simulink model "Sistema1"  (R2026a)
settings: Solver=ode15s  StopTime=20  MaxStep=0.01  RelTol=1e-6
libraries: fl_lib x18, nesl_utility x6, slpidlib x1
settings Model: Creator=sarag  LastModifiedBy=emivilg
settings DataIOCC: TimeSaveName=t
settings SimscapeCC: SimscapeNominalValues="[{\"value\":\"1\",\"unit\":\"A\"},{\"value\":\"1\",\"unit\":\"bar\"},{\"value\":\"1\",\"unit\":\"cm^2\"},{\"value\":\"1\",\"unit\":\"cm^3/s\"},{\"value\":\"1\",\"unit\":\"kJ/kg\"},{\"value\":\"1\",\"unit\":\"kW\"},{\"value\":\"1\",\"unit\":\"l\"},{\"value\":\"1\",\"unit\":\"N\"},{\"value\":\"1\",\"unit\":\"N*m\"},{\"value\":\"1\",\"unit\":\"V\"}]"  SimscapeLogType=none  SimscapeLogDataHistory=5000.0

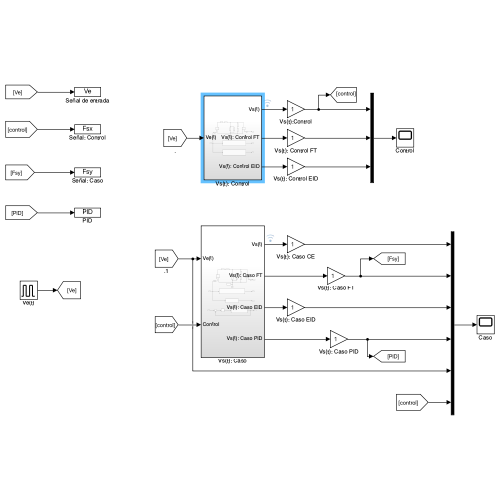
[thumbnail: Simulink's stored preview of the top-level diagram]
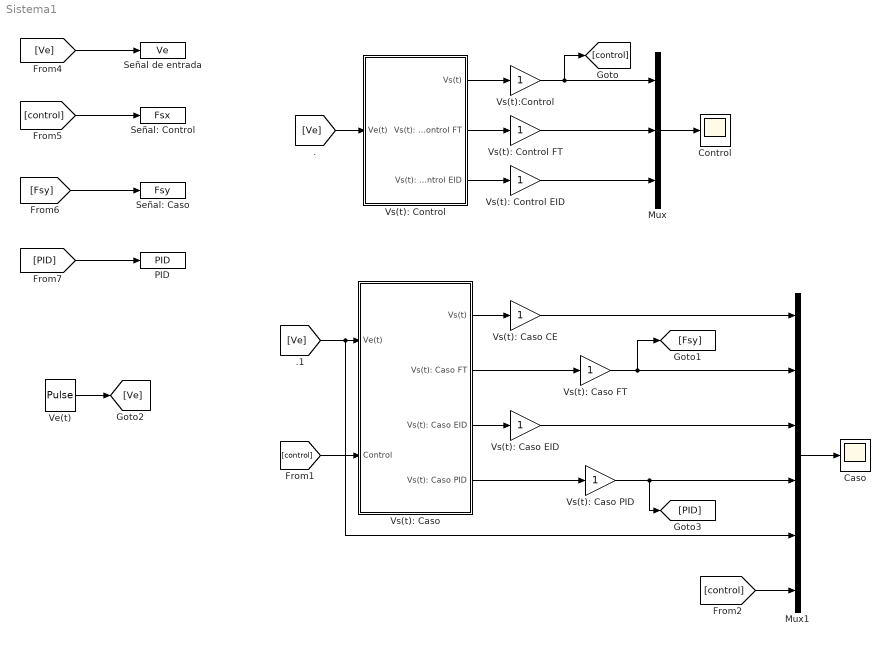
== system Sistema1 ==
  Caso : Scope
      settings: ActiveDisplayYMinimum=-0.12376243766517554  ActiveDisplayYMaximum=1.1138614462905658
  Control : Scope
      settings: ActiveDisplayYMinimum=-0.12361899608688497  ActiveDisplayYMaximum=1.112570964781965
  Mux : Mux  Inputs=3
  Mux1 : Mux  Inputs=6
  PID : ToWorkspace  VariableName=PID  SampleTime=-1
  Señal de entrada : ToWorkspace  VariableName=Ve  SampleTime=-1
  Señal: Caso : ToWorkspace  VariableName=Fsy  SampleTime=-1
  Señal: Control : ToWorkspace  VariableName=Fsx  SampleTime=-1
  Ve(t) : DiscretePulseGenerator  PulseType=Time based  Period=10  PulseWidth=5
  Vs(t): Caso : Subsystem
  Vs(t): Caso CE : Gain
  Vs(t): Caso EID : Gain
  Vs(t): Caso FT : Gain
  Vs(t): Caso PID : Gain
  Vs(t): Control : Subsystem
  Vs(t): Control EID : Gain
  Vs(t): Control FT : Gain
  Vs(t):Control : Gain
  wires:
  Mux/1 -> Control/1
  [Ve] -> Vs(t): Control/1(Ve(t))
  Vs(t): Control/1(Vs(t)) -> Vs(t):Control/1
  Vs(t): Caso/1(Vs(t)) -> Vs(t): Caso CE/1
  Vs(t): Caso/2(Vs(t): Caso FT) -> Vs(t): Caso FT/1
  Vs(t): Caso/3(Vs(t): Caso EID) -> Vs(t): Caso EID/1
  Vs(t): Caso/4(Vs(t): Caso PID) -> Vs(t): Caso PID/1
  Mux1/1 -> Caso/1
  Vs(t): Control/2(Vs(t): Control FT) -> Vs(t): Control FT/1
  Vs(t): Control/3(Vs(t): Control EID) -> Vs(t): Control EID/1
  Ve(t)/1 -> [Ve]
  [PID] -> PID/1
  [Fsy] -> Señal: Caso/1
  [control] -> Señal: Control/1
  [Ve] -> Señal de entrada/1
  Vs(t):Control/1 -> [control], Mux/1
  Vs(t): Control EID/1 -> Mux/3
  Vs(t): Caso CE/1 -> Mux1/1
  Vs(t): Caso FT/1 -> [Fsy], Mux1/2
  Vs(t): Caso EID/1 -> Mux1/3
  Vs(t): Caso PID/1 -> [PID], Mux1/4
  [control] -> Vs(t): Caso/2(Control)
  Vs(t): Control FT/1 -> Mux/2
  [control] -> Mux1/6
  [Ve] -> Mux1/5, Vs(t): Caso/1(Ve(t))

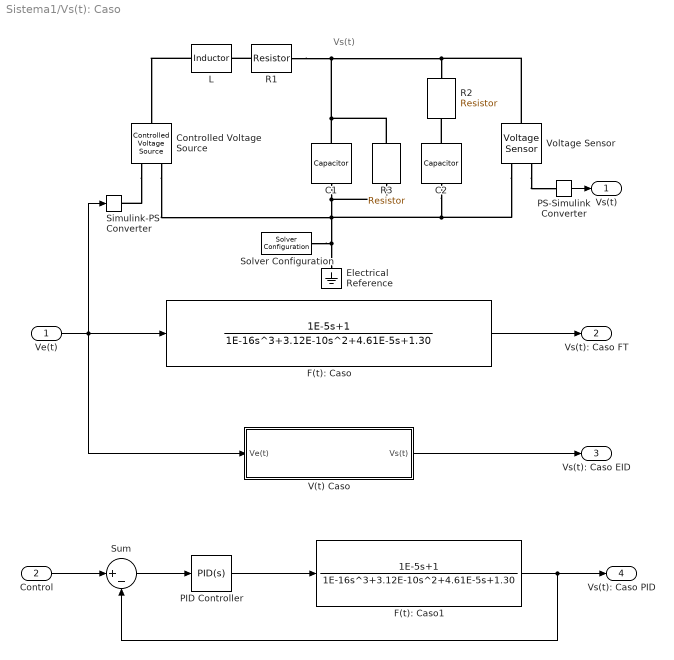
== system Sistema1/Vs(t): Caso ==
  note: Vs(t)
  Ve(t) : Inport
  Control : Inport  Port=2
  C1 : fl_lib/Electrical/Electrical Elements/Capacitor  c=1 uF  r=1e-6 Ohm  g=0 1/Ohm  i_specify=off  i_priority=None  i=0 A  i_nominal_specify=off  i_nominal_value=1  i_nominal_unit=A  v_specify=off  v_priority=None  v=0 V  v_nominal_specify=off  v_nominal_value=1  v_nominal_unit=V  vc_specify=off  vc_priority=High  vc=0 V  vc_nominal_specify=off  vc_nominal_value=1  vc_nominal_unit=V
  C2 : fl_lib/Electrical/Electrical Elements/Capacitor  c=0.1 uF  r=1e-6 Ohm  g=0 1/Ohm  i_specify=off  i_priority=None  i=0 A  i_nominal_specify=off  i_nominal_value=1  i_nominal_unit=A  v_specify=off  v_priority=None  v=0 V  v_nominal_specify=off  v_nominal_value=1  v_nominal_unit=V  vc_specify=off  vc_priority=High  vc=0 V  vc_nominal_specify=off  vc_nominal_value=1  vc_nominal_unit=V
  Controlled Voltage Source : fl_lib/Electrical/Electrical Sources/Controlled Voltage Source
  Electrical Reference : fl_lib/Electrical/Electrical Elements/Electrical Reference
  F(t): Caso : TransferFcn  Numerator=[1E-5, 1]  Denominator=[1E-16, 3.12E-10, 4.61E-5, 1.30 ]
  F(t): Caso1 : TransferFcn  Numerator=[1E-5, 1]  Denominator=[1E-16, 3.12E-10, 4.61E-5, 1.30 ]
  L : fl_lib/Electrical/Electrical Elements/Inductor  l=10 uH  r=0 Ohm  g=1e-9 1/Ohm  i_specify=off  i_priority=None  i=0 A  i_nominal_specify=off  i_nominal_value=1  i_nominal_unit=A  v_specify=off  v_priority=None  v=0 V  v_nominal_specify=off  v_nominal_value=1  v_nominal_unit=V  i_L_specify=off  i_L_priority=High  i_L=0 A  i_L_nominal_specify=off  i_L_nominal_value=1  i_L_nominal_unit=A
  PID Controller : slpidlib/PID Controller  Controller=PID  Form=Parallel  TimeDomain=Continuous-time  UseExternalTs=off  SampleTime=-1  IntegratorMethod=Forward Euler  FilterMethod=Forward Euler  ControllerParametersSource=internal  P=0.703106505048227  I=25112.1670097634  UseKiTs=off  D=-4.39908221517028e-06  UseExternalDerivativeSource=off  N=23788.0653667222  UseFilter=on  TunerSelectOption=Transfer Function Based (PID Tuner App)  InitialConditionSource=internal  InitialConditionForIntegrator=0  InitialConditionForFilter=0  DifferentiatorICPrevScaledInput=0  ExternalReset=none  TrackingMode=off  Kt=1  LimitOutput=off  SatLimitsSource=internal  UpperSaturationLimit=inf  LowerSaturationLimit=-inf  LinearizeAsGain=on  AntiWindupMode=none  Kb=1  LimitIntegrator=off  UpperIntegratorSaturationLimit=inf  LowerIntegratorSaturationLimit=-inf  POutMin=[]  POutMax=[]  IOutMin=[]  IOutMax=[]  DOutMin=[]  DOutMax=[]  NOutMin=[]  NOutMax=[]  SumOutMin=[]  SumOutMax=[]  SaturationOutMin=[]  SaturationOutMax=[]  PParamMin=[]  PParamMax=[]  IParamMin=[]  IParamMax=[]  DParamMin=[]  DParamMax=[]  NParamMin=[]  NParamMax=[]  KbParamMin=[]  KbParamMax=[]  KtParamMin=[]  KtParamMax=[]  KbOutMin=[]  KbOutMax=[]  KtOutMin=[]  KtOutMax=[]  IntegratorOutMin=[]  IntegratorOutMax=[]  FilterOutMin=[]  FilterOutMax=[]  SumI1OutMin=[]  SumI1OutMax=[]  SumI2OutMin=[]  SumI2OutMax=[]  SumI3OutMin=[]  SumI3OutMax=[]  SumI4OutMin=[]  SumI4OutMax=[]  SumDOutMin=[]  SumDOutMax=[]  DifferentiatorOutMin=[]  DifferentiatorOutMax=[]  FilterDiffOutCoefMin=[]  FilterDiffOutCoefMax=[]  ReciprocalOutMin=[]  ReciprocalOutMax=[]  SumDenOutMin=[]  SumDenOutMax=[]  SumNumOutMin=[]  SumNumOutMax=[]  DivideOutMin=[]  DivideOutMax=[]  UdiffTsProdOutMin=[]  UdiffTsProdOutMax=[]  NTsProdOutMin=[]  NTsProdOutMax=[]  UintegralTsProdOutMin=[]  UintegralTsProdOutMax=[]  UngainTsProdOutMin=[]  UngainTsProdOutMax=[]  ClampingZeroOutDataTypeStr=Inherit: Inherit via back propagation  ClampingZeroOutMin=[]  ClampingZeroOutMax=[]  FilterDenConstantOutDataTypeStr=Inherit: Inherit via back propagation  FilterDenConstantOutMin=[]  FilterDenConstantOutMax=[]  PCopyOutDataTypeStr=Inherit: Inherit via back propagation  PCopyOutMin=[]  PCopyOutMax=[]  NCopyOutDataTypeStr=Inherit: Inherit via back propagation  NCopyOutMin=[]  NCopyOutMax=[]  IntegratorContinuousStateAttributes=''  IntegratorStateMustResolveToSignalObject=off  IntegratorRTWStateStorageClass=Auto  FilterContinuousStateAttributes=''  FilterStateMustResolveToSignalObject=off  FilterRTWStateStorageClass=Auto  ParallelPVariant=InternalParameters  IdealPVariant=Disabled  IVariant=InternalParameters  DVariant=InternalParameters  IntegratorVariant=Continuous  SatVariant=Disabled  AWVariant=Passthrough  PCopyVariant=Disabled  TRVariant=Disabled  FdbkBlocksVariant=Forward  IdealPFdbkVariant=Disabled  SatFdbkVariant=Disabled  DerivativeFilterVariant=ContFilter  NVariant=InternalParameters  NCopyVariant=Disabled  FilterICVariant=InternalICsFilter  IntegratorICVariant=InternalICs  ExternalResetVariant=Disabled  TRSumVariant=Passthrough  SumFdbkVariant=Disabled  SumVariant=Sum_PID  TsampFilterVariant=InternalTs  TsampNgainVariant=Passthrough  TsampIntegralVariant=Disabled_SignalSpec  ExternalSaturationOutDataTypeStr=Inherit: Same as second input  DerivativeSourceVariant=ErrorSignal  PreIntVariant=InternalPreInt
  PS-Simulink Converter : nesl_utility/PS-Simulink Converter  PhysicalDomain=network_engine_domain  SubClassName=ps_output  LeftPortType=input  RightPortType=output  PseudoPeriodic=off  Frequencies=[]  VectorFormat=inherit  Unit=inherit  AffineConversion=off
  R1 : fl_lib/Electrical/Electrical Elements/Resistor  R=30 Ohm  i_specify=off  i_priority=None  i=0 A  i_nominal_specify=off  i_nominal_value=1  i_nominal_unit=A  v_specify=off  v_priority=None  v=0 V  v_nominal_specify=off  v_nominal_value=1  v_nominal_unit=V
  R2 : fl_lib/Electrical/Electrical Elements/Resistor  R=100 Ohm  i_specify=off  i_priority=None  i=0 A  i_nominal_specify=off  i_nominal_value=1  i_nominal_unit=A  v_specify=off  v_priority=None  v=0 V  v_nominal_specify=off  v_nominal_value=1  v_nominal_unit=V
  R3 : fl_lib/Electrical/Electrical Elements/Resistor  R=100 Ohm  i_specify=off  i_priority=None  i=0 A  i_nominal_specify=off  i_nominal_value=1  i_nominal_unit=A  v_specify=off  v_priority=None  v=0 V  v_nominal_specify=off  v_nominal_value=1  v_nominal_unit=V
  Simulink-PS Converter : nesl_utility/Simulink-PS Converter  PhysicalDomain=network_engine_domain  SubClassName=ps_input  LeftPortType=input  RightPortType=output  PseudoPeriodic=off  Frequencies=[]  NoiseDistribution=none  NoiseParameters=[]  Unit=1  AffineConversion=off  FilteringAndDerivatives=provide  SimscapeFilterOrder=1  InputFilterTimeConstant=0.001  UdotUserProvided=0
  Solver Configuration : nesl_utility/Solver Configuration  PhysicalDomain=network_engine_domain  SubClassName=solver  LeftPortType=input  RightPortType=generic  Tones=[]  Harmonics=[]  SimulateNoise=off  Profile=off  UseLocalSampling=off  EnableSwitchedLinearOptims=on  FrequencyDomain=off  UseCCode=off  RelTol=0.001  AbsTol=0.001  MinStep=1e-09  ToWorkspace=off  RevertToSquareIcSolve=off  NumHomotopyIterations=100  PhasorMode=off  PhasorModeNumHarmonics=1  ConsistencySolver=NEWTON_XTOL_AFTER_FTOL  CanonicalOrdering=UNORDERED  OptimizeIntermediates=UNOPTIMIZED  IndexReductionMethod=DerivativeReplacement  DoDC=off  ResidualTolerance=1e-09  ConsistencyTolSource=GLOBAL  ConsistencyAbsTol=0.001  ConsistencyRelTol=0.001  ConsistencyTolFactor=0.001  UseLocalSolver=off  LocalSolverChoice=NE_BACKWARD_EULER_ADVANCER  ResolveIndetEquations=on  FunctionEvalNumThread=1  LocalSolverSampleTime=0.001  DoFixedCost=off  MaxNonlinIter=3  MaxModeIter=2  ComputeImpulses=off  ImpulseIterations=2  LinearAlgebra=auto  LinearAlgebraNumThread=0  EquationFormulation=NE_TIME_EF  DelaysMemoryBudget=1024  AutomaticFiltering=on  FilteringTimeConstant=0.001  PartitionStorageMethod=AS_NEEDED  PartitionMemoryBudget=1024  PartitionMethod=ROBUST  MultibodyUseLocalSolver=off  MultibodyLocalSolverChoice=ODE1  MultibodyLocalSolverSampleTime=0.001
  Sum : Sum  Inputs=|+-
  V(t) Caso : Subsystem
  Voltage Sensor : fl_lib/Electrical/Electrical Sensors/Voltage Sensor
  Vs(t) : Outport
  Vs(t): Caso FT : Outport  Port=2
  Vs(t): Caso EID : Outport  Port=3
  Vs(t): Caso PID : Outport  Port=4
  wires:
  PS-Simulink Converter/1 -> Vs(t)/1
  F(t): Caso/1 -> Vs(t): Caso FT/1
  Control/1 -> Sum/1
  PID Controller/1 -> F(t): Caso1/1
  Sum/1 -> PID Controller/1
  F(t): Caso1/1 -> Vs(t): Caso PID/1, Sum/2
  Ve(t)/1 -> V(t) Caso/1(Ve(t)), Simulink-PS Converter/1, F(t): Caso/1
  V(t) Caso/1(Vs(t)) -> Vs(t): Caso EID/1
  connections:
  Voltage Sensor/LConn1 -- R2/LConn1 -- R1/RConn1 -- C1/LConn1 -- R3/LConn1
  R3/RConn1 -- C1/RConn1 -- Controlled Voltage Source/RConn2 -- Solver Configuration/RConn1 -- Electrical Reference/LConn1 -- Voltage Sensor/RConn2 -- C2/RConn1
  Voltage Sensor/RConn1 -- PS-Simulink Converter/LConn1
  Controlled Voltage Source/RConn1 -- Simulink-PS Converter/RConn1
  R1/LConn1 -- L/RConn1
  L/LConn1 -- Controlled Voltage Source/LConn1
  C2/LConn1 -- R2/RConn1

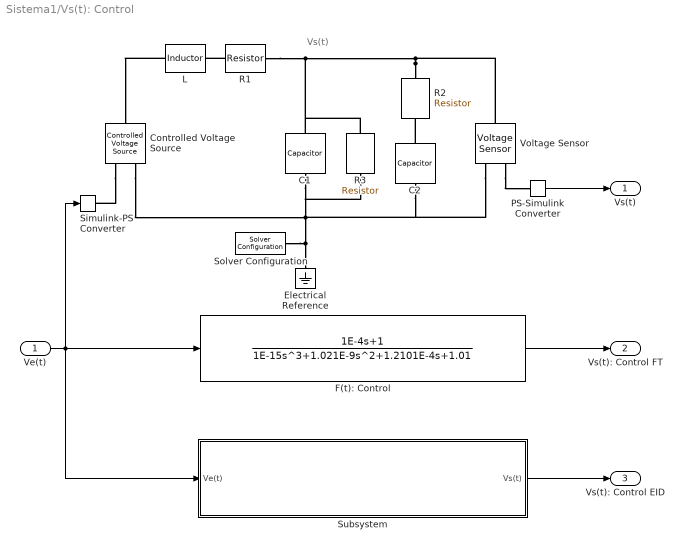
== system Sistema1/Vs(t): Control ==
  note: Vs(t)
  Ve(t) : Inport
  C1 : fl_lib/Electrical/Electrical Elements/Capacitor  c=1 uF  r=1e-6 Ohm  g=0 1/Ohm  i_specify=off  i_priority=None  i=0 A  i_nominal_specify=off  i_nominal_value=1  i_nominal_unit=A  v_specify=off  v_priority=None  v=0 V  v_nominal_specify=off  v_nominal_value=1  v_nominal_unit=V  vc_specify=off  vc_priority=High  vc=0 V  vc_nominal_specify=off  vc_nominal_value=1  vc_nominal_unit=V
  C2 : fl_lib/Electrical/Electrical Elements/Capacitor  c=1 uF  r=1e-6 Ohm  g=0 1/Ohm  i_specify=off  i_priority=None  i=0 A  i_nominal_specify=off  i_nominal_value=1  i_nominal_unit=A  v_specify=off  v_priority=None  v=0 V  v_nominal_specify=off  v_nominal_value=1  v_nominal_unit=V  vc_specify=off  vc_priority=High  vc=0 V  vc_nominal_specify=off  vc_nominal_value=1  vc_nominal_unit=V
  Controlled Voltage Source : fl_lib/Electrical/Electrical Sources/Controlled Voltage Source
  Electrical Reference : fl_lib/Electrical/Electrical Elements/Electrical Reference
  F(t): Control : TransferFcn  Numerator=[1E-4, 1]  Denominator=[1E-15, 1.021E-9, 1.2101E-4, 1.01 ]
  L : fl_lib/Electrical/Electrical Elements/Inductor  l=10 uH  r=0 Ohm  g=1e-9 1/Ohm  i_specify=off  i_priority=None  i=0 A  i_nominal_specify=off  i_nominal_value=1  i_nominal_unit=A  v_specify=off  v_priority=None  v=0 V  v_nominal_specify=off  v_nominal_value=1  v_nominal_unit=V  i_L_specify=off  i_L_priority=High  i_L=0 A  i_L_nominal_specify=off  i_L_nominal_value=1  i_L_nominal_unit=A
  PS-Simulink Converter : nesl_utility/PS-Simulink Converter  PhysicalDomain=network_engine_domain  SubClassName=ps_output  LeftPortType=input  RightPortType=output  PseudoPeriodic=off  Frequencies=[]  VectorFormat=inherit  Unit=inherit  AffineConversion=off
  R1 : fl_lib/Electrical/Electrical Elements/Resistor  R=10 Ohm  i_specify=off  i_priority=None  i=0 A  i_nominal_specify=off  i_nominal_value=1  i_nominal_unit=A  v_specify=off  v_priority=None  v=0 V  v_nominal_specify=off  v_nominal_value=1  v_nominal_unit=V
  R2 : fl_lib/Electrical/Electrical Elements/Resistor  R=100 Ohm  i_specify=off  i_priority=None  i=0 A  i_nominal_specify=off  i_nominal_value=1  i_nominal_unit=A  v_specify=off  v_priority=None  v=0 V  v_nominal_specify=off  v_nominal_value=1  v_nominal_unit=V
  R3 : fl_lib/Electrical/Electrical Elements/Resistor  R=1 kOhm  i_specify=off  i_priority=None  i=0 A  i_nominal_specify=off  i_nominal_value=1  i_nominal_unit=A  v_specify=off  v_priority=None  v=0 V  v_nominal_specify=off  v_nominal_value=1  v_nominal_unit=V
  Simulink-PS Converter : nesl_utility/Simulink-PS Converter  PhysicalDomain=network_engine_domain  SubClassName=ps_input  LeftPortType=input  RightPortType=output  PseudoPeriodic=off  Frequencies=[]  NoiseDistribution=none  NoiseParameters=[]  Unit=1  AffineConversion=off  FilteringAndDerivatives=provide  SimscapeFilterOrder=1  InputFilterTimeConstant=0.001  UdotUserProvided=0
  Solver Configuration : nesl_utility/Solver Configuration  PhysicalDomain=network_engine_domain  SubClassName=solver  LeftPortType=input  RightPortType=generic  Tones=[]  Harmonics=[]  SimulateNoise=off  Profile=off  UseLocalSampling=off  EnableSwitchedLinearOptims=on  FrequencyDomain=off  UseCCode=off  RelTol=0.001  AbsTol=0.001  MinStep=1e-09  ToWorkspace=off  RevertToSquareIcSolve=off  NumHomotopyIterations=100  PhasorMode=off  PhasorModeNumHarmonics=1  ConsistencySolver=NEWTON_XTOL_AFTER_FTOL  CanonicalOrdering=UNORDERED  OptimizeIntermediates=UNOPTIMIZED  IndexReductionMethod=DerivativeReplacement  DoDC=off  ResidualTolerance=1e-09  ConsistencyTolSource=GLOBAL  ConsistencyAbsTol=0.001  ConsistencyRelTol=0.001  ConsistencyTolFactor=0.001  UseLocalSolver=off  LocalSolverChoice=NE_BACKWARD_EULER_ADVANCER  ResolveIndetEquations=on  FunctionEvalNumThread=1  LocalSolverSampleTime=0.001  DoFixedCost=off  MaxNonlinIter=3  MaxModeIter=2  ComputeImpulses=off  ImpulseIterations=2  LinearAlgebra=auto  LinearAlgebraNumThread=0  EquationFormulation=NE_TIME_EF  DelaysMemoryBudget=1024  AutomaticFiltering=on  FilteringTimeConstant=0.001  PartitionStorageMethod=AS_NEEDED  PartitionMemoryBudget=1024  PartitionMethod=ROBUST  MultibodyUseLocalSolver=off  MultibodyLocalSolverChoice=ODE1  MultibodyLocalSolverSampleTime=0.001
  Subsystem : Subsystem
  Voltage Sensor : fl_lib/Electrical/Electrical Sensors/Voltage Sensor
  Vs(t) : Outport
  Vs(t): Control FT : Outport  Port=2
  Vs(t): Control EID : Outport  Port=3
  wires:
  PS-Simulink Converter/1 -> Vs(t)/1
  Ve(t)/1 -> Subsystem/1(Ve(t)), Simulink-PS Converter/1, F(t): Control/1
  F(t): Control/1 -> Vs(t): Control FT/1
  Subsystem/1(Vs(t)) -> Vs(t): Control EID/1
  connections:
  R2/LConn1 -- R3/LConn1 -- C1/LConn1 -- R1/RConn1 -- Voltage Sensor/LConn1
  Controlled Voltage Source/RConn2 -- C2/RConn1 -- Voltage Sensor/RConn2 -- R3/RConn1 -- C1/RConn1 -- Solver Configuration/RConn1 -- Electrical Reference/LConn1
  Voltage Sensor/RConn1 -- PS-Simulink Converter/LConn1
  Controlled Voltage Source/RConn1 -- Simulink-PS Converter/RConn1
  R1/LConn1 -- L/RConn1
  L/LConn1 -- Controlled Voltage Source/LConn1
  C2/LConn1 -- R2/RConn1

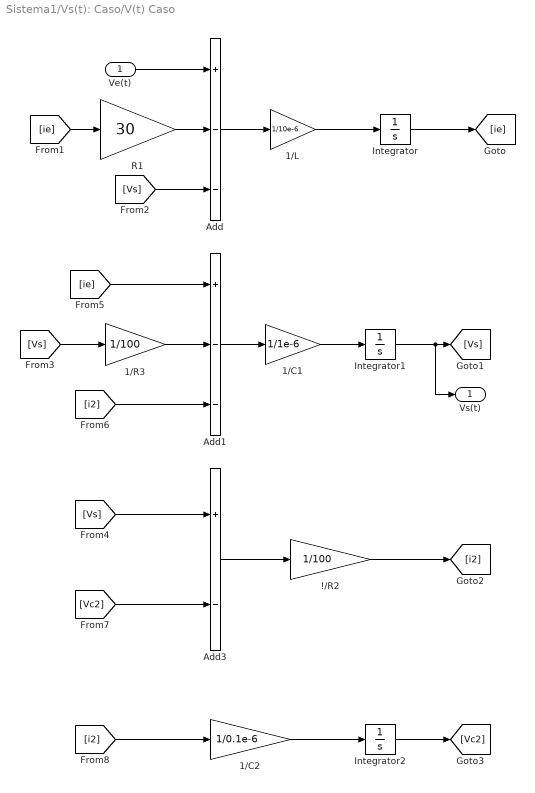
== system Sistema1/Vs(t): Caso/V(t) Caso ==
  Ve(t) : Inport
  !/R2 : Gain  Gain=1/100
  1/C1 : Gain  Gain=1/1e-6
  1/C2 : Gain  Gain=1/0.1e-6
  1/L : Gain  Gain=1/10e-6
  1/R3 : Gain  Gain=1/100
  Add : Sum  Inputs=+--
  Add1 : Sum  Inputs=+--
  Add3 : Sum  Inputs=+-
  Integrator : Integrator
  Integrator1 : Integrator
  Integrator2 : Integrator
  R1 : Gain  Gain=30
  Vs(t) : Outport
  wires:
  !/R2/1 -> [i2]
  [ie] -> R1/1
  Integrator2/1 -> [Vc2]
  [Vs] -> Add/3
  Add1/1 -> 1/C1/1
  Ve(t)/1 -> Add/1
  Integrator/1 -> [ie]
  1/C1/1 -> Integrator1/1
  [i2] -> 1/C2/1
  [Vs] -> 1/R3/1
  [Vc2] -> Add3/2
  1/C2/1 -> Integrator2/1
  1/L/1 -> Integrator/1
  R1/1 -> Add/2
  [ie] -> Add1/1
  Integrator1/1 -> Vs(t)/1, [Vs]
  [Vs] -> Add3/1
  1/R3/1 -> Add1/2
  [i2] -> Add1/3
  Add/1 -> 1/L/1
  Add3/1 -> !/R2/1

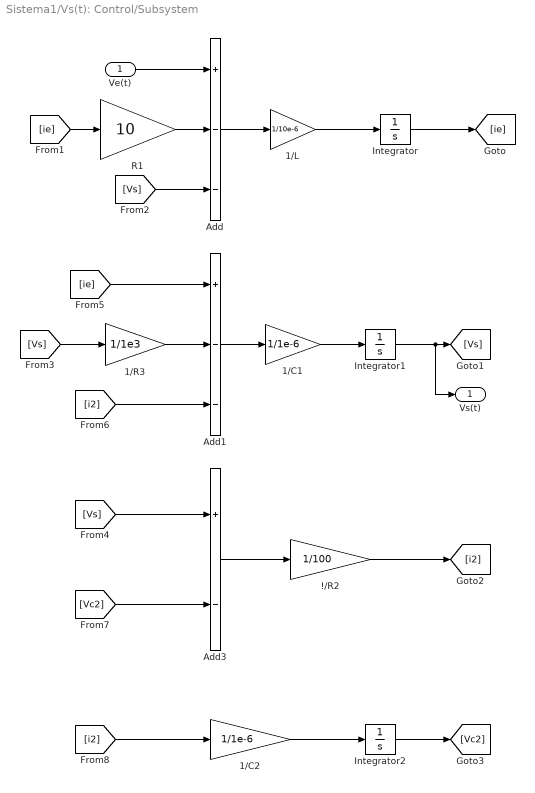
== system Sistema1/Vs(t): Control/Subsystem ==
  Ve(t) : Inport
  !/R2 : Gain  Gain=1/100
  1/C1 : Gain  Gain=1/1e-6
  1/C2 : Gain  Gain=1/1e-6
  1/L : Gain  Gain=1/10e-6
  1/R3 : Gain  Gain=1/1e3
  Add : Sum  Inputs=+--
  Add1 : Sum  Inputs=+--
  Add3 : Sum  Inputs=+-
  Integrator : Integrator
  Integrator1 : Integrator
  Integrator2 : Integrator
  R1 : Gain  Gain=10
  Vs(t) : Outport
  wires:
  !/R2/1 -> [i2]
  [ie] -> R1/1
  [Vs] -> Add/3
  Ve(t)/1 -> Add/1
  [Vc2] -> Add3/2
  1/C1/1 -> Integrator1/1
  [Vs] -> 1/R3/1
  Integrator1/1 -> Vs(t)/1, [Vs]
  [Vs] -> Add3/1
  R1/1 -> Add/2
  1/L/1 -> Integrator/1
  1/R3/1 -> Add1/2
  Add1/1 -> 1/C1/1
  [i2] -> Add1/3
  Add/1 -> 1/L/1
  [ie] -> Add1/1
  Integrator2/1 -> [Vc2]
  Add3/1 -> !/R2/1
  Integrator/1 -> [ie]
  1/C2/1 -> Integrator2/1
  [i2] -> 1/C2/1
